simulink model "sst_cllc_dcx"  (R2026b)
settings: Solver=ode23tb  StopTime=param.sim.simlength  FixedStep=tc  MaxStep=param.glb_time.tc
values from neighbouring files (symbols this model uses):
  param = struct()    [init_model.m]
undefined symbols (not defined in the file or in its folder): cllc_dcx_param_example
libraries: fl_lib x144, nesl_utility x71, mos_simple_2th_lib x8, discrete_time_low_pass_filter x2, lithium_ion_battery x1, cllc_dcx x1, single_phase_transformer x1, dab_single_phase_pwm_modulator x1, ee_lib x1
(part 2 of 4)

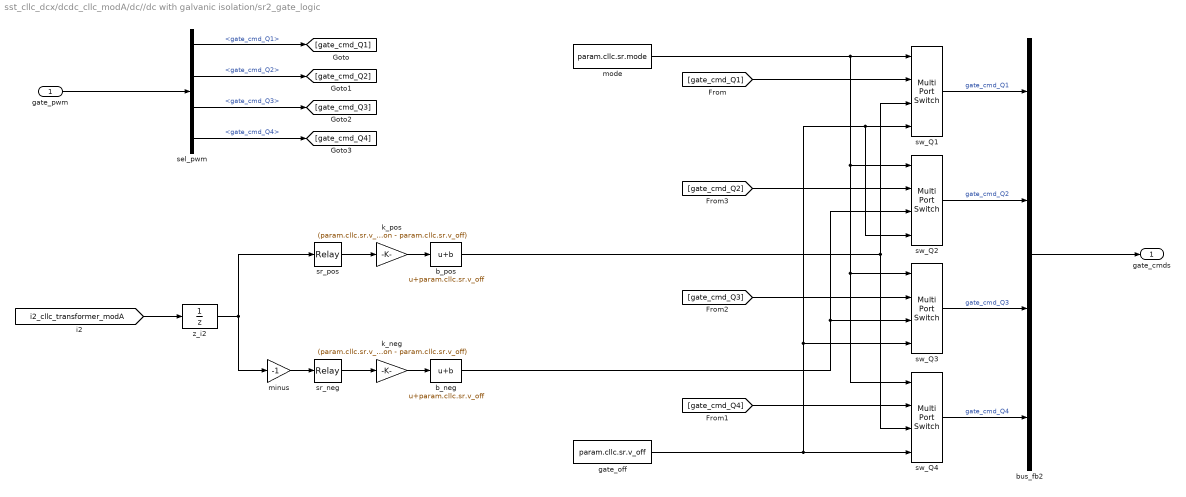
== system sst_cllc_dcx/dcdc_cllc_modA/dc//dc with galvanic isolation/sr2_gate_logic ==
  gate_pwm : Inport
  b_neg : Bias  Bias=param.cllc.sr.v_off  SaturateOnIntegerOverflow=off
  b_pos : Bias  Bias=param.cllc.sr.v_off  SaturateOnIntegerOverflow=off
  bus_fb2 : BusCreator  Inputs=4
  gate_off : Constant  Value=param.cllc.sr.v_off
  k_neg : Gain  Gain=(param.cllc.sr.v_on - param.cllc.sr.v_off)
  k_pos : Gain  Gain=(param.cllc.sr.v_on - param.cllc.sr.v_off)
  minus : Gain  Gain=-1
  mode : Constant  Value=param.cllc.sr.mode
  sel_pwm : BusSelector  OutputSignals=gate_cmd_Q1,gate_cmd_Q2,gate_cmd_Q3,gate_cmd_Q4
  sr_neg : Relay  OnSwitchValue=param.cllc.sr.i_on  OffSwitchValue=param.cllc.sr.i_off
  sr_pos : Relay  OnSwitchValue=param.cllc.sr.i_on  OffSwitchValue=param.cllc.sr.i_off
  sw_Q{1..4} (4 alike) : MultiPortSwitch  DataPortOrder=Zero-based contiguous  zeroidx=on  SaturateOnIntegerOverflow=off  InputSameDT=off
  z_i2 : UnitDelay  SampleTime=param.glb_time.tc
  gate_cmds : Outport
  wires:
  gate_pwm/1 -> sel_pwm/1
  [i2_cllc_transformer_modA] -> z_i2/1
  z_i2/1 -> sr_pos/1, minus/1
  minus/1 -> sr_neg/1
  sr_pos/1 -> k_pos/1
  k_pos/1 -> b_pos/1
  sr_neg/1 -> k_neg/1
  k_neg/1 -> b_neg/1
  mode/1 -> sw_Q1/1, sw_Q2/1, sw_Q3/1, sw_Q4/1
  [gate_cmd_Q1] -> sw_Q1/2
  b_pos/1 -> sw_Q4/3, sw_Q1/3
  gate_off/1 -> sw_Q3/4, sw_Q1/4, sw_Q2/4, sw_Q4/4
  sw_Q1/1 -> bus_fb2/1  "gate_cmd_Q1"
  [gate_cmd_Q2] -> sw_Q2/2
  b_neg/1 -> sw_Q3/3, sw_Q2/3
  sw_Q2/1 -> bus_fb2/2  "gate_cmd_Q2"
  [gate_cmd_Q3] -> sw_Q3/2
  sw_Q3/1 -> bus_fb2/3  "gate_cmd_Q3"
  [gate_cmd_Q4] -> sw_Q4/2
  sw_Q4/1 -> bus_fb2/4  "gate_cmd_Q4"
  bus_fb2/1 -> gate_cmds/1
  sel_pwm/1 -> [gate_cmd_Q1]  "<gate_cmd_Q1>"
  sel_pwm/2 -> [gate_cmd_Q2]  "<gate_cmd_Q2>"
  sel_pwm/3 -> [gate_cmd_Q3]  "<gate_cmd_Q3>"
  sel_pwm/4 -> [gate_cmd_Q4]  "<gate_cmd_Q4>"

== system sst_cllc_dcx/dcdc_cllc_modA/input_current_control/input_current_control ==
  current_input_pu : Inport
  local_time : Inport  Port=2
  Trigger : TriggerPort  VariantControl=(inherit)  PortDimensions=1
  Gain : Gain  Gain=-1
  Gain1 : Gain  Gain=-1
  LLC_current_input_tracking : Scope  NumInputPorts=4
      settings: ActiveDisplayYMinimum=-0.41147300652049457  ActiveDisplayYMaximum=1.0697728708256782  DataLoggingVariableName=ScopeData12
  Quantizer : Quantizer  QuantizationInterval=param.meas.adc12_quantization
  Step : Step  InitialValue=1  FinalValue=-1
  To Workspace1 : ToWorkspace  VariableName=cllc_input_current_ref_sim  SampleTime=-1
      settings: MaxDataPoints=param.glb_time.Ns_cllc
  To Workspace14 : ToWorkspace  VariableName=time_ts_sim  SampleTime=-1
      settings: MaxDataPoints=param.glb_time.Ns_cllc
  To Workspace2 : ToWorkspace  VariableName=cllc_input_current_sim  SampleTime=-1
      settings: MaxDataPoints=param.glb_time.Ns_cllc
  To Workspace3 : ToWorkspace  VariableName=cllc_current_ctrl_output_sim  SampleTime=-1
      settings: MaxDataPoints=param.glb_time.Ns_cllc
  Unit Delay2 : UnitDelay  SampleTime=-1
  Zero-Order Hold1 : ZeroOrderHold  SampleTime=-1
  Zero-Order Hold2 : ZeroOrderHold  SampleTime=-1
  current_control : Subsystem
  discrete-time-low-pass-filter : discrete_time_low_pass_filter/discrete-time-low-pass-filter  tau=0.025  ts=param.glb_time.ts_cllc
  discrete-time-low-pass-filter1 : discrete_time_low_pass_filter/discrete-time-low-pass-filter  tau=0.025  ts=param.glb_time.ts_cllc
  ictrl_out : Outport
  wires:
  Unit Delay2/1 -> To Workspace3/1, LLC_current_input_tracking/3, ictrl_out/1  "current_ctrl_output"
  current_control/1(ctrli_out) -> Gain/1
  Quantizer/1 -> Zero-Order Hold2/1
  current_input_pu/1 -> Quantizer/1
  Zero-Order Hold2/1 -> LLC_current_input_tracking/2, To Workspace2/1, current_control/2(iout), LLC_current_input_tracking/4  "i_dc_input"
  Gain/1 -> Unit Delay2/1
  local_time/1 -> Zero-Order Hold1/1
  Zero-Order Hold1/1 -> To Workspace14/1
  Step/1 -> Gain1/1
  discrete-time-low-pass-filter/1 -> LLC_current_input_tracking/1, To Workspace1/1, current_control/1(iout_ref)  "current_input_ref"
  Gain1/1 -> discrete-time-low-pass-filter/1

== system sst_cllc_dcx/dcdc_cllc_modA/input_current_control/modulator ==
  phase_displacement : Inport
  Constant1 : Constant  Value=0.5
  Constant2 : Constant  Value=0.5
  Constant3 : Constant  Value=0.02
  dab_single_phase_pwm_modulator : dab_single_phase_pwm_modulator/dab_single_phase_pwm_modulator  fPWM_DAB=param.glb_time.fPWM_CLLC  m_up=1  m_low=0  dead_time_DAB=param.glb_time.dead_time_CLLC  pos_cmd_gate=18  neg_cmd_gate=-3  polarity=-1  tc=param.glb_time.tc  max_phase_displacement=pi/2  trgo_double_update=param.glb_time.TRGO_CLLC_double_update
  gate_cmds : Outport
  tag scope: TRGO=global
  wires:
  dab_single_phase_pwm_modulator/2 -> gate_cmds/1
  Constant2/1 -> dab_single_phase_pwm_modulator/3
  dab_single_phase_pwm_modulator/1 -> [TRGO]
  Constant1/1 -> dab_single_phase_pwm_modulator/2
  [time_cllc_module_1] -> dab_single_phase_pwm_modulator/1
  Constant3/1 -> dab_single_phase_pwm_modulator/4

== system sst_cllc_dcx/dcdc_cllc_modA/input_current_control/normalization ==
  in : Inport
  1/Ti3 : Gain  Gain=1/param.cllc.hw.Idc_FS  OutDataTypeStr=double  SaturateOnIntegerOverflow=on  ParamDataTypeStr=Inherit: Same as input
  out_pu : Outport
  wires:
  in/1 -> 1/Ti3/1
  1/Ti3/1 -> out_pu/1

== system sst_cllc_dcx/dcdc_cllc_modA/dc//dc with galvanic isolation/full-bridge 1/full-full_bridge_ssc_mosfet_based ==
  gate_commands : Inport
  data_measure : Subsystem
  full_bridge_ssc_mosfet_based : Subsystem  mask{mass_heatsink_m=param.thermal.heatsink.no_weight, specific_heat_m=param.thermal.heatsink.cp, rth_mosfet_HA_m=param.thermal.heatsink.Rth_mosfet_HA, rth_mosfet_JH_m=param.cllc.mosfet.Rth_mosfet_JH, Rds_on_m=param.cllc.mosfet.Rds_on, Vth_m=param.cllc.mosfet.Vth, Eon_m=param.cllc.mosfet.Eon, Eoff_m=param.cllc.mosfet.Eoff, Voff_sw_loss_m=param.cllc.mosfet.Voff_sw_losses, Ion_sw_loss_m=param.cllc.mosfet.Ion_sw_losses, Vdon_diode_m=param.cllc.mosfet.Vdon_diode, Rdon_diode_m=param.cllc.mosfet.Rds_on, JunctionTermalMass_m=param.cllc.mosfet.JunctionTermalMass, Tambient_m=param.thermal.Tambient, DThs_init_m=param.thermal.DThs_init, Csnubber_m=param.cllc.mosfet.Csnubber_zvs, Rsnubber_m=param.cllc.mosfet.Rsnubber_zvs}
      mask prompts: mass_heatsink_m "Mass Heatsink (kg)"; specific_heat_m "Specific Heat (J/K/kg)"; rth_mosfet_HA_m "Thermal Resistance HA (K/W)"; rth_mosfet_JH_m "Thermal Resistance JH (K/W)"; Rds_on_m "Rds_on (Ohm)"; Vth_m "Vth (V)"; Eon_m "Eon (J)"; Eoff_m "Eoff (J)"; Voff_sw_loss_m "Voff_sw_loss (V)"; Ion_sw_loss_m "Ion_sw_loss (A)"; Vdon_diode_m "Vdon_diode (V)"; Rdon_diode_m "Rdon_diode (Ohm)"; JunctionTermalMass_m "JunctionTermalMass (J/K)"; Tambient_m "Tambient (degC)"; DThs_init_m "DThs_init (degC)"; Csnubber_m "Csnubber (F)"; Rsnubber_m "Rsnubber (Ohm)"
  udc(+) : PMIOPort  Side=Left
  udc(-) : PMIOPort  Port=2  Side=Left
  uac(+) : PMIOPort  Port=3  Side=Right
  uac(-) : PMIOPort  Port=4  Side=Right
  wires:
  full_bridge_ssc_mosfet_based/1(m) -> data_measure/1(m)
  gate_commands/1 -> full_bridge_ssc_mosfet_based/1(gate_commands)
  connections:
  full_bridge_ssc_mosfet_based/LConn2 -- udc(-)/RConn1
  full_bridge_ssc_mosfet_based/LConn1 -- udc(+)/RConn1
  full_bridge_ssc_mosfet_based/RConn2 -- uac(-)/RConn1
  full_bridge_ssc_mosfet_based/RConn1 -- uac(+)/RConn1

== system sst_cllc_dcx/dcdc_cllc_modA/dc//dc with galvanic isolation/full-bridge 2/full_bridge_ssc_mosfet_based ==
  gate_commands : Inport
  data_measure : Subsystem
  full_bridge_ssc_mosfet_based : Subsystem  mask{mass_heatsink_m=param.thermal.heatsink.no_weight, specific_heat_m=param.thermal.heatsink.cp, rth_mosfet_HA_m=param.thermal.heatsink.Rth_mosfet_HA, rth_mosfet_JH_m=param.cllc.mosfet_sr.Rth_mosfet_JH, Rds_on_m=param.cllc.mosfet_sr.Rds_on, Vth_m=param.cllc.mosfet_sr.Vth, Eon_m=param.cllc.mosfet_sr.Eon, Eoff_m=param.cllc.mosfet_sr.Eoff, Voff_sw_loss_m=param.cllc.mosfet_sr.Voff_sw_losses, Ion_sw_loss_m=param.cllc.mosfet_sr.Ion_sw_losses, Vdon_diode_m=param.cllc.mosfet_sr.Vdon_diode, Rdon_diode_m=param.cllc.mosfet_sr.Rds_on, JunctionTermalMass_m=param.cllc.mosfet_sr.JunctionTermalMass, Tambient_m=param.thermal.Tambient, DThs_init_m=param.thermal.DThs_init, Csnubber_m=param.cllc.mosfet_sr.Csnubber_zvs, Rsnubber_m=param.cllc.mosfet_sr.Rsnubber_zvs}
      mask prompts: mass_heatsink_m "Mass Heatsink (kg)"; specific_heat_m "Specific Heat (J/K/kg)"; rth_mosfet_HA_m "Thermal Resistance HA (K/W)"; rth_mosfet_JH_m "Thermal Resistance JH (K/W)"; Rds_on_m "Rds_on (Ohm)"; Vth_m "Vth (V)"; Eon_m "Eon (J)"; Eoff_m "Eoff (J)"; Voff_sw_loss_m "Voff_sw_loss (V)"; Ion_sw_loss_m "Ion_sw_loss (A)"; Vdon_diode_m "Vdon_diode (V)"; Rdon_diode_m "Rdon_diode (Ohm)"; JunctionTermalMass_m "JunctionTermalMass (J/K)"; Tambient_m "Tambient (degC)"; DThs_init_m "DThs_init (degC)"; Csnubber_m "Csnubber (F)"; Rsnubber_m "Rsnubber (Ohm)"
  udc(+) : PMIOPort  Side=Left
  udc(-) : PMIOPort  Port=2  Side=Left
  uac(+) : PMIOPort  Port=3  Side=Right
  uac(-) : PMIOPort  Port=4  Side=Right
  wires:
  full_bridge_ssc_mosfet_based/1(m) -> data_measure/1(m)
  gate_commands/1 -> full_bridge_ssc_mosfet_based/1(gate_commands)
  connections:
  full_bridge_ssc_mosfet_based/LConn2 -- udc(-)/RConn1
  full_bridge_ssc_mosfet_based/LConn1 -- udc(+)/RConn1
  full_bridge_ssc_mosfet_based/RConn2 -- uac(-)/RConn1
  full_bridge_ssc_mosfet_based/RConn1 -- uac(+)/RConn1

== system sst_cllc_dcx/dcdc_cllc_modA/input_current_control/input_current_control/current_control ==
  iout_ref : Inport
  iout : Inport  Port=2
  Sum2 : Sum  Inputs=+-  OutDataTypeStr=double  AccumDataTypeStr=double  SaturateOnIntegerOverflow=on
  iout_ctrl : Subsystem
  ctrli_out : Outport
  wires:
  iout_ctrl/1(phase_shift) -> ctrli_out/1
  iout/1 -> Sum2/2
  iout_ref/1 -> Sum2/1
  Sum2/1 -> iout_ctrl/1(i_tilde)

== system sst_cllc_dcx/dcdc_cllc_modA/dc//dc with galvanic isolation/full-bridge 1/full-full_bridge_ssc_mosfet_based/data_measure ==
  m : Inport
  Bus Selector : BusSelector  OutputSignals=mosfet_ploss_Q1,mosfet_voltage_Q1,mosfet_current_Q1,mosfet_JH_temp_Q1,mosfet_HA_temp_Q1
  Bus Selector1 : BusSelector  OutputSignals=mosfet_ploss_Q2,mosfet_voltage_Q2,mosfet_current_Q2,mosfet_JH_temp_Q2,mosfet_HA_temp_Q2
  tag scope: inverter_1_cllc_mosfet_zvs_modA=global, mosfet_zvs_HA_temp_cllc_Q1=global, mosfet_zvs_HA_temp_cllc_Q2=global, mosfet_zvs_JH_temp_cllc_Q1=global, mosfet_zvs_JH_temp_cllc_Q2=global, mosfet_zvs_ids_cllc_Q1=global, mosfet_zvs_ids_cllc_Q2=global, mosfet_zvs_plosses_cllc_Q1=global, mosfet_zvs_plosses_cllc_Q2=global, mosfet_zvs_uds_cllc_Q1=global, mosfet_zvs_uds_cllc_Q2=global
  wires:
  Bus Selector/1 -> [mosfet_zvs_plosses_cllc_Q1]  "<mosfet_ploss_Q1>"
  Bus Selector1/3 -> [mosfet_zvs_ids_cllc_Q2]  "<mosfet_current_Q2>"
  Bus Selector1/2 -> [mosfet_zvs_uds_cllc_Q2]  "<mosfet_voltage_Q2>"
  Bus Selector1/5 -> [mosfet_zvs_HA_temp_cllc_Q2]  "<mosfet_HA_temp_Q2>"
  Bus Selector/4 -> [mosfet_zvs_JH_temp_cllc_Q1]  "<mosfet_JH_temp_Q1>"
  Bus Selector/5 -> [mosfet_zvs_HA_temp_cllc_Q1]  "<mosfet_HA_temp_Q1>"
  Bus Selector1/4 -> [mosfet_zvs_JH_temp_cllc_Q2]  "<mosfet_JH_temp_Q2>"
  Bus Selector/3 -> [mosfet_zvs_ids_cllc_Q1]  "<mosfet_current_Q1>"
  Bus Selector/2 -> [mosfet_zvs_uds_cllc_Q1]  "<mosfet_voltage_Q1>"
  Bus Selector1/1 -> [mosfet_zvs_plosses_cllc_Q2]  "<mosfet_ploss_Q2>"
  m/1 -> Bus Selector/1, Bus Selector1/1, [inverter_1_cllc_mosfet_zvs_modA]

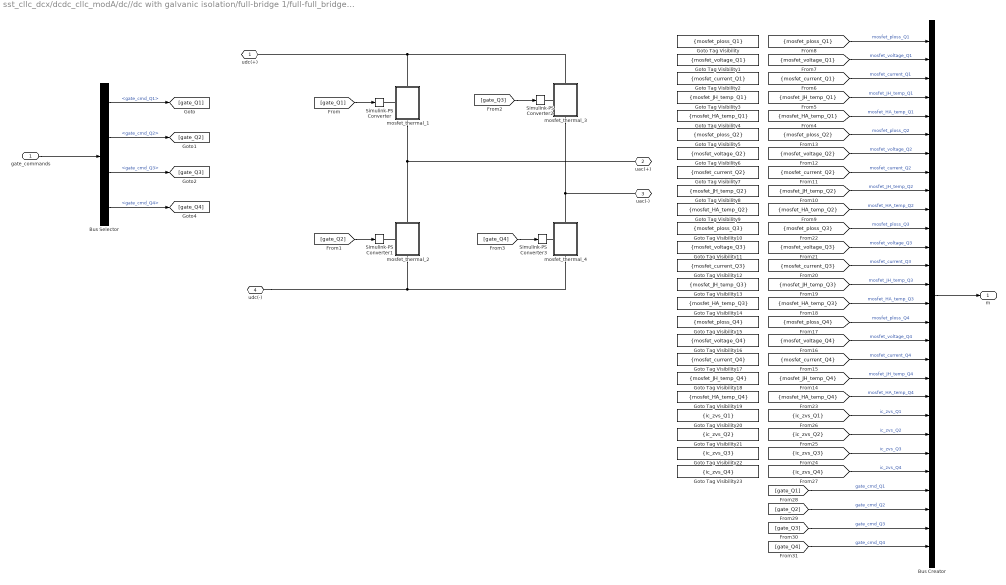
== system sst_cllc_dcx/dcdc_cllc_modA/dc//dc with galvanic isolation/full-bridge 1/full-full_bridge_ssc_mosfet_based/full_bridge_ssc_mosfet_based ==
  gate_commands : Inport
  Bus Creator : BusCreator  Inputs=28
  Bus Selector : BusSelector  OutputSignals=gate_cmd_Q1,gate_cmd_Q2,gate_cmd_Q3,gate_cmd_Q4
  Goto Tag Visibility : GotoTagVisibility  GotoTag=mosfet_ploss_Q1
  Goto Tag Visibility1 : GotoTagVisibility  GotoTag=mosfet_voltage_Q1
  Goto Tag Visibility10 : GotoTagVisibility  GotoTag=mosfet_ploss_Q3
  Goto Tag Visibility11 : GotoTagVisibility  GotoTag=mosfet_voltage_Q3
  Goto Tag Visibility12 : GotoTagVisibility  GotoTag=mosfet_current_Q3
  Goto Tag Visibility13 : GotoTagVisibility  GotoTag=mosfet_JH_temp_Q3
  Goto Tag Visibility14 : GotoTagVisibility  GotoTag=mosfet_HA_temp_Q3
  Goto Tag Visibility15 : GotoTagVisibility  GotoTag=mosfet_ploss_Q4
  Goto Tag Visibility16 : GotoTagVisibility  GotoTag=mosfet_voltage_Q4
  Goto Tag Visibility17 : GotoTagVisibility  GotoTag=mosfet_current_Q4
  Goto Tag Visibility18 : GotoTagVisibility  GotoTag=mosfet_JH_temp_Q4
  Goto Tag Visibility19 : GotoTagVisibility  GotoTag=mosfet_HA_temp_Q4
  Goto Tag Visibility2 : GotoTagVisibility  GotoTag=mosfet_current_Q1
  Goto Tag Visibility20 : GotoTagVisibility  GotoTag=ic_zvs_Q1
  Goto Tag Visibility21 : GotoTagVisibility  GotoTag=ic_zvs_Q2
  Goto Tag Visibility22 : GotoTagVisibility  GotoTag=ic_zvs_Q3
  Goto Tag Visibility23 : GotoTagVisibility  GotoTag=ic_zvs_Q4
  Goto Tag Visibility3 : GotoTagVisibility  GotoTag=mosfet_JH_temp_Q1
  Goto Tag Visibility4 : GotoTagVisibility  GotoTag=mosfet_HA_temp_Q1
  Goto Tag Visibility5 : GotoTagVisibility  GotoTag=mosfet_ploss_Q2
  Goto Tag Visibility6 : GotoTagVisibility  GotoTag=mosfet_voltage_Q2
  Goto Tag Visibility7 : GotoTagVisibility  GotoTag=mosfet_current_Q2
  Goto Tag Visibility8 : GotoTagVisibility  GotoTag=mosfet_JH_temp_Q2
  Goto Tag Visibility9 : GotoTagVisibility  GotoTag=mosfet_HA_temp_Q2
  Simulink-PS Converter{,1..3} (4 alike) : nesl_utility/Simulink-PS Converter  PhysicalDomain=network_engine_domain  SubClassName=ps_input  LeftPortType=input  RightPortType=output  PseudoPeriodic=off  Frequencies=[]  NoiseDistribution=none  NoiseParameters=[]  Unit=V  AffineConversion=off  FilteringAndDerivatives=provide  SimscapeFilterOrder=1  InputFilterTimeConstant=0.001  UdotUserProvided=0
  mosfet_thermal_1 : Subsystem
      settings: PortSchema="{\"entries\":[{\"content\":{\"sides\":[{\"content\":{\"connectorIds\":[\"LConn1\"]},\"type\":\"ConnectorPlacement.EquallySpacedRectSide\",\"uuid\":\"9277da8d-d460-43e6-8478-dd662f15d226\"},{\"content\":{\"connectorIds\":[],\"side\":\"RIGHT\"},\"type\":\"ConnectorPlacement.EquallySpacedRectSide\",\"uuid\":\"a7ece396-f1d9-4f4f-a05b-db1fc65d6e1d\"},{\"content\":{\"connectorIds\":[\"LConn2\"],\"side\":\"TOP\"},\"type\":\"ConnectorPlacement.EquallySpacedRectSide\",\"uuid\":\"fdd70777-e9cf-4317-afb6-cae87f75d5b0\"},{\"content\":{\"connectorIds\":[\"RConn1\"],\"side\":\"BOTTOM\"},\"type\":\"ConnectorPlacement.EquallySpacedRectSide\",\"uuid\":\"2353ed68-b1a1-4775-9ca9-31e268d5443b\"}]},\"type\":\"ConnectorPlacement.EquallySpacedConnector\",\"uuid\":\"d5479f4c-4e65-4791-adcb-73df11f88590\"}],\"packageUris\":[\"http://schema.mathworks.com/mf0/Connector/R2020b\"],\"version\":\"1.0\"}"
  mosfet_thermal_2 : Subsystem
      settings: PortSchema="{\"entries\":[{\"content\":{\"sides\":[{\"content\":{\"connectorIds\":[\"LConn1\"]},\"type\":\"ConnectorPlacement.EquallySpacedRectSide\",\"uuid\":\"9277da8d-d460-43e6-8478-dd662f15d226\"},{\"content\":{\"connectorIds\":[],\"side\":\"RIGHT\"},\"type\":\"ConnectorPlacement.EquallySpacedRectSide\",\"uuid\":\"a7ece396-f1d9-4f4f-a05b-db1fc65d6e1d\"},{\"content\":{\"connectorIds\":[\"LConn2\"],\"side\":\"TOP\"},\"type\":\"ConnectorPlacement.EquallySpacedRectSide\",\"uuid\":\"fdd70777-e9cf-4317-afb6-cae87f75d5b0\"},{\"content\":{\"connectorIds\":[\"RConn1\"],\"side\":\"BOTTOM\"},\"type\":\"ConnectorPlacement.EquallySpacedRectSide\",\"uuid\":\"2353ed68-b1a1-4775-9ca9-31e268d5443b\"}]},\"type\":\"ConnectorPlacement.EquallySpacedConnector\",\"uuid\":\"d5479f4c-4e65-4791-adcb-73df11f88590\"}],\"packageUris\":[\"http://schema.mathworks.com/mf0/Connector/R2020b\"],\"version\":\"1.0\"}"
  mosfet_thermal_3 : Subsystem
      settings: PortSchema="{\"entries\":[{\"content\":{\"sides\":[{\"content\":{\"connectorIds\":[\"LConn1\"]},\"type\":\"ConnectorPlacement.EquallySpacedRectSide\",\"uuid\":\"9277da8d-d460-43e6-8478-dd662f15d226\"},{\"content\":{\"connectorIds\":[],\"side\":\"RIGHT\"},\"type\":\"ConnectorPlacement.EquallySpacedRectSide\",\"uuid\":\"a7ece396-f1d9-4f4f-a05b-db1fc65d6e1d\"},{\"content\":{\"connectorIds\":[\"LConn2\"],\"side\":\"TOP\"},\"type\":\"ConnectorPlacement.EquallySpacedRectSide\",\"uuid\":\"fdd70777-e9cf-4317-afb6-cae87f75d5b0\"},{\"content\":{\"connectorIds\":[\"RConn1\"],\"side\":\"BOTTOM\"},\"type\":\"ConnectorPlacement.EquallySpacedRectSide\",\"uuid\":\"2353ed68-b1a1-4775-9ca9-31e268d5443b\"}]},\"type\":\"ConnectorPlacement.EquallySpacedConnector\",\"uuid\":\"d5479f4c-4e65-4791-adcb-73df11f88590\"}],\"packageUris\":[\"http://schema.mathworks.com/mf0/Connector/R2020b\"],\"version\":\"1.0\"}"
  mosfet_thermal_4 : Subsystem
      settings: PortSchema="{\"entries\":[{\"content\":{\"sides\":[{\"content\":{\"connectorIds\":[\"LConn1\"]},\"type\":\"ConnectorPlacement.EquallySpacedRectSide\",\"uuid\":\"9277da8d-d460-43e6-8478-dd662f15d226\"},{\"content\":{\"connectorIds\":[],\"side\":\"RIGHT\"},\"type\":\"ConnectorPlacement.EquallySpacedRectSide\",\"uuid\":\"a7ece396-f1d9-4f4f-a05b-db1fc65d6e1d\"},{\"content\":{\"connectorIds\":[\"LConn2\"],\"side\":\"TOP\"},\"type\":\"ConnectorPlacement.EquallySpacedRectSide\",\"uuid\":\"fdd70777-e9cf-4317-afb6-cae87f75d5b0\"},{\"content\":{\"connectorIds\":[\"RConn1\"],\"side\":\"BOTTOM\"},\"type\":\"ConnectorPlacement.EquallySpacedRectSide\",\"uuid\":\"2353ed68-b1a1-4775-9ca9-31e268d5443b\"}]},\"type\":\"ConnectorPlacement.EquallySpacedConnector\",\"uuid\":\"d5479f4c-4e65-4791-adcb-73df11f88590\"}],\"packageUris\":[\"http://schema.mathworks.com/mf0/Connector/R2020b\"],\"version\":\"1.0\"}"
  udc(+) : PMIOPort  Side=Left
  uac(+) : PMIOPort  Port=2  Side=Right
  uac(-) : PMIOPort  Port=3  Side=Right
  udc(-) : PMIOPort  Port=4  Side=Left
  m : Outport
  wires:
  [gate_Q4] -> Bus Creator/28  "gate_cmd_Q4"
  [gate_Q3] -> Bus Creator/27  "gate_cmd_Q3"
  [gate_Q2] -> Bus Creator/26  "gate_cmd_Q2"
  [gate_Q1] -> Bus Creator/25  "gate_cmd_Q1"
  [ic_zvs_Q4] -> Bus Creator/24  "ic_zvs_Q4"
  [ic_zvs_Q3] -> Bus Creator/23  "ic_zvs_Q3"
  [ic_zvs_Q2] -> Bus Creator/22  "ic_zvs_Q2"
  [ic_zvs_Q1] -> Bus Creator/21  "ic_zvs_Q1"
  Bus Creator/1 -> m/1
  [mosfet_HA_temp_Q4] -> Bus Creator/20  "mosfet_HA_temp_Q4"
  [mosfet_JH_temp_Q4] -> Bus Creator/19  "mosfet_JH_temp_Q4"
  [mosfet_current_Q4] -> Bus Creator/18  "mosfet_current_Q4"
  [mosfet_voltage_Q4] -> Bus Creator/17  "mosfet_voltage_Q4"
  [mosfet_ploss_Q4] -> Bus Creator/16  "mosfet_ploss_Q4"
  [mosfet_HA_temp_Q3] -> Bus Creator/15  "mosfet_HA_temp_Q3"
  [mosfet_JH_temp_Q3] -> Bus Creator/14  "mosfet_JH_temp_Q3"
  [mosfet_current_Q3] -> Bus Creator/13  "mosfet_current_Q3"
  [mosfet_voltage_Q3] -> Bus Creator/12  "mosfet_voltage_Q3"
  [mosfet_ploss_Q3] -> Bus Creator/11  "mosfet_ploss_Q3"
  [mosfet_HA_temp_Q2] -> Bus Creator/10  "mosfet_HA_temp_Q2"
  [mosfet_JH_temp_Q2] -> Bus Creator/9  "mosfet_JH_temp_Q2"
  [mosfet_current_Q2] -> Bus Creator/8  "mosfet_current_Q2"
  [mosfet_voltage_Q2] -> Bus Creator/7  "mosfet_voltage_Q2"
  [mosfet_ploss_Q2] -> Bus Creator/6  "mosfet_ploss_Q2"
  [mosfet_HA_temp_Q1] -> Bus Creator/5  "mosfet_HA_temp_Q1"
  [mosfet_JH_temp_Q1] -> Bus Creator/4  "mosfet_JH_temp_Q1"
  [mosfet_current_Q1] -> Bus Creator/3  "mosfet_current_Q1"
  [mosfet_voltage_Q1] -> Bus Creator/2  "mosfet_voltage_Q1"
  [mosfet_ploss_Q1] -> Bus Creator/1  "mosfet_ploss_Q1"
  [gate_Q3] -> Simulink-PS Converter2/1
  Bus Selector/2 -> [gate_Q2]  "<gate_cmd_Q2>"
  Bus Selector/1 -> [gate_Q1]  "<gate_cmd_Q1>"
  Bus Selector/3 -> [gate_Q3]  "<gate_cmd_Q3>"
  [gate_Q4] -> Simulink-PS Converter3/1
  [gate_Q2] -> Simulink-PS Converter1/1
  [gate_Q1] -> Simulink-PS Converter/1
  Bus Selector/4 -> [gate_Q4]  "<gate_cmd_Q4>"
  gate_commands/1 -> Bus Selector/1
  connections:
  mosfet_thermal_1/LConn1 -- Simulink-PS Converter/RConn1
  mosfet_thermal_3/LConn2 -- udc(+)/RConn1 -- mosfet_thermal_1/LConn2
  mosfet_thermal_4/RConn1 -- udc(-)/RConn1 -- mosfet_thermal_2/RConn1
  mosfet_thermal_2/LConn2 -- mosfet_thermal_1/RConn1 -- uac(+)/RConn1
  mosfet_thermal_3/LConn1 -- Simulink-PS Converter2/RConn1
  mosfet_thermal_4/LConn2 -- uac(-)/RConn1 -- mosfet_thermal_3/RConn1
  mosfet_thermal_2/LConn1 -- Simulink-PS Converter1/RConn1
  mosfet_thermal_4/LConn1 -- Simulink-PS Converter3/RConn1

== system sst_cllc_dcx/dcdc_cllc_modA/dc//dc with galvanic isolation/full-bridge 2/full_bridge_ssc_mosfet_based/data_measure ==
  m : Inport
  Bus Selector : BusSelector  OutputSignals=mosfet_ploss_Q1,mosfet_voltage_Q1,mosfet_current_Q1,mosfet_JH_temp_Q1,mosfet_HA_temp_Q1
  Bus Selector1 : BusSelector  OutputSignals=mosfet_ploss_Q2,mosfet_voltage_Q2,mosfet_current_Q2,mosfet_JH_temp_Q2,mosfet_HA_temp_Q2
  tag scope: inverter_2_cllc_mosfet_zvs_modA=global, mosfet_zvs_HA_temp_cllc_Q5=global, mosfet_zvs_HA_temp_cllc_Q6=global, mosfet_zvs_JH_temp_cllc_Q5=global, mosfet_zvs_JH_temp_cllc_Q6=global, mosfet_zvs_ids_cllc_Q5=global, mosfet_zvs_ids_cllc_Q6=global, mosfet_zvs_plosses_cllc_Q5=global, mosfet_zvs_plosses_cllc_Q6=global, mosfet_zvs_uds_cllc_Q5=global, mosfet_zvs_uds_cllc_Q6=global
  wires:
  Bus Selector/1 -> [mosfet_zvs_plosses_cllc_Q5]  "<mosfet_ploss_Q1>"
  Bus Selector1/3 -> [mosfet_zvs_ids_cllc_Q6]  "<mosfet_current_Q2>"
  Bus Selector1/2 -> [mosfet_zvs_uds_cllc_Q6]  "<mosfet_voltage_Q2>"
  Bus Selector1/5 -> [mosfet_zvs_HA_temp_cllc_Q6]  "<mosfet_HA_temp_Q2>"
  Bus Selector/4 -> [mosfet_zvs_JH_temp_cllc_Q5]  "<mosfet_JH_temp_Q1>"
  Bus Selector/5 -> [mosfet_zvs_HA_temp_cllc_Q5]  "<mosfet_HA_temp_Q1>"
  Bus Selector1/4 -> [mosfet_zvs_JH_temp_cllc_Q6]  "<mosfet_JH_temp_Q2>"
  Bus Selector/3 -> [mosfet_zvs_ids_cllc_Q5]  "<mosfet_current_Q1>"
  Bus Selector/2 -> [mosfet_zvs_uds_cllc_Q5]  "<mosfet_voltage_Q1>"
  Bus Selector1/1 -> [mosfet_zvs_plosses_cllc_Q6]  "<mosfet_ploss_Q2>"
  m/1 -> Bus Selector/1, Bus Selector1/1, [inverter_2_cllc_mosfet_zvs_modA]

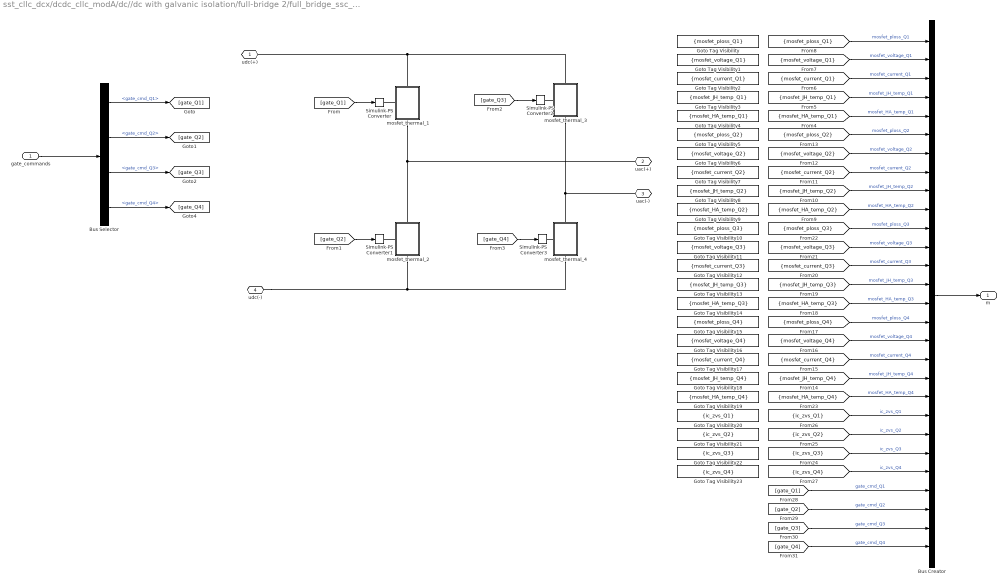
== system sst_cllc_dcx/dcdc_cllc_modA/dc//dc with galvanic isolation/full-bridge 2/full_bridge_ssc_mosfet_based/full_bridge_ssc_mosfet_based ==
  gate_commands : Inport
  Bus Creator : BusCreator  Inputs=28
  Bus Selector : BusSelector  OutputSignals=gate_cmd_Q1,gate_cmd_Q2,gate_cmd_Q3,gate_cmd_Q4
  Goto Tag Visibility : GotoTagVisibility  GotoTag=mosfet_ploss_Q1
  Goto Tag Visibility1 : GotoTagVisibility  GotoTag=mosfet_voltage_Q1
  Goto Tag Visibility10 : GotoTagVisibility  GotoTag=mosfet_ploss_Q3
  Goto Tag Visibility11 : GotoTagVisibility  GotoTag=mosfet_voltage_Q3
  Goto Tag Visibility12 : GotoTagVisibility  GotoTag=mosfet_current_Q3
  Goto Tag Visibility13 : GotoTagVisibility  GotoTag=mosfet_JH_temp_Q3
  Goto Tag Visibility14 : GotoTagVisibility  GotoTag=mosfet_HA_temp_Q3
  Goto Tag Visibility15 : GotoTagVisibility  GotoTag=mosfet_ploss_Q4
  Goto Tag Visibility16 : GotoTagVisibility  GotoTag=mosfet_voltage_Q4
  Goto Tag Visibility17 : GotoTagVisibility  GotoTag=mosfet_current_Q4
  Goto Tag Visibility18 : GotoTagVisibility  GotoTag=mosfet_JH_temp_Q4
  Goto Tag Visibility19 : GotoTagVisibility  GotoTag=mosfet_HA_temp_Q4
  Goto Tag Visibility2 : GotoTagVisibility  GotoTag=mosfet_current_Q1
  Goto Tag Visibility20 : GotoTagVisibility  GotoTag=ic_zvs_Q1
  Goto Tag Visibility21 : GotoTagVisibility  GotoTag=ic_zvs_Q2
  Goto Tag Visibility22 : GotoTagVisibility  GotoTag=ic_zvs_Q3
  Goto Tag Visibility23 : GotoTagVisibility  GotoTag=ic_zvs_Q4
  Goto Tag Visibility3 : GotoTagVisibility  GotoTag=mosfet_JH_temp_Q1
  Goto Tag Visibility4 : GotoTagVisibility  GotoTag=mosfet_HA_temp_Q1
  Goto Tag Visibility5 : GotoTagVisibility  GotoTag=mosfet_ploss_Q2
  Goto Tag Visibility6 : GotoTagVisibility  GotoTag=mosfet_voltage_Q2
  Goto Tag Visibility7 : GotoTagVisibility  GotoTag=mosfet_current_Q2
  Goto Tag Visibility8 : GotoTagVisibility  GotoTag=mosfet_JH_temp_Q2
  Goto Tag Visibility9 : GotoTagVisibility  GotoTag=mosfet_HA_temp_Q2
  Simulink-PS Converter{,1..3} (4 alike) : nesl_utility/Simulink-PS Converter  PhysicalDomain=network_engine_domain  SubClassName=ps_input  LeftPortType=input  RightPortType=output  PseudoPeriodic=off  Frequencies=[]  NoiseDistribution=none  NoiseParameters=[]  Unit=V  AffineConversion=off  FilteringAndDerivatives=provide  SimscapeFilterOrder=1  InputFilterTimeConstant=0.001  UdotUserProvided=0
  mosfet_thermal_1 : Subsystem
      settings: PortSchema="{\"entries\":[{\"content\":{\"sides\":[{\"content\":{\"connectorIds\":[\"LConn1\"]},\"type\":\"ConnectorPlacement.EquallySpacedRectSide\",\"uuid\":\"9277da8d-d460-43e6-8478-dd662f15d226\"},{\"content\":{\"connectorIds\":[],\"side\":\"RIGHT\"},\"type\":\"ConnectorPlacement.EquallySpacedRectSide\",\"uuid\":\"a7ece396-f1d9-4f4f-a05b-db1fc65d6e1d\"},{\"content\":{\"connectorIds\":[\"LConn2\"],\"side\":\"TOP\"},\"type\":\"ConnectorPlacement.EquallySpacedRectSide\",\"uuid\":\"fdd70777-e9cf-4317-afb6-cae87f75d5b0\"},{\"content\":{\"connectorIds\":[\"RConn1\"],\"side\":\"BOTTOM\"},\"type\":\"ConnectorPlacement.EquallySpacedRectSide\",\"uuid\":\"2353ed68-b1a1-4775-9ca9-31e268d5443b\"}]},\"type\":\"ConnectorPlacement.EquallySpacedConnector\",\"uuid\":\"d5479f4c-4e65-4791-adcb-73df11f88590\"}],\"packageUris\":[\"http://schema.mathworks.com/mf0/Connector/R2020b\"],\"version\":\"1.0\"}"
  mosfet_thermal_2 : Subsystem
      settings: PortSchema="{\"entries\":[{\"content\":{\"sides\":[{\"content\":{\"connectorIds\":[\"LConn1\"]},\"type\":\"ConnectorPlacement.EquallySpacedRectSide\",\"uuid\":\"9277da8d-d460-43e6-8478-dd662f15d226\"},{\"content\":{\"connectorIds\":[],\"side\":\"RIGHT\"},\"type\":\"ConnectorPlacement.EquallySpacedRectSide\",\"uuid\":\"a7ece396-f1d9-4f4f-a05b-db1fc65d6e1d\"},{\"content\":{\"connectorIds\":[\"LConn2\"],\"side\":\"TOP\"},\"type\":\"ConnectorPlacement.EquallySpacedRectSide\",\"uuid\":\"fdd70777-e9cf-4317-afb6-cae87f75d5b0\"},{\"content\":{\"connectorIds\":[\"RConn1\"],\"side\":\"BOTTOM\"},\"type\":\"ConnectorPlacement.EquallySpacedRectSide\",\"uuid\":\"2353ed68-b1a1-4775-9ca9-31e268d5443b\"}]},\"type\":\"ConnectorPlacement.EquallySpacedConnector\",\"uuid\":\"d5479f4c-4e65-4791-adcb-73df11f88590\"}],\"packageUris\":[\"http://schema.mathworks.com/mf0/Connector/R2020b\"],\"version\":\"1.0\"}"
  mosfet_thermal_3 : Subsystem
      settings: PortSchema="{\"entries\":[{\"content\":{\"sides\":[{\"content\":{\"connectorIds\":[\"LConn1\"]},\"type\":\"ConnectorPlacement.EquallySpacedRectSide\",\"uuid\":\"9277da8d-d460-43e6-8478-dd662f15d226\"},{\"content\":{\"connectorIds\":[],\"side\":\"RIGHT\"},\"type\":\"ConnectorPlacement.EquallySpacedRectSide\",\"uuid\":\"a7ece396-f1d9-4f4f-a05b-db1fc65d6e1d\"},{\"content\":{\"connectorIds\":[\"LConn2\"],\"side\":\"TOP\"},\"type\":\"ConnectorPlacement.EquallySpacedRectSide\",\"uuid\":\"fdd70777-e9cf-4317-afb6-cae87f75d5b0\"},{\"content\":{\"connectorIds\":[\"RConn1\"],\"side\":\"BOTTOM\"},\"type\":\"ConnectorPlacement.EquallySpacedRectSide\",\"uuid\":\"2353ed68-b1a1-4775-9ca9-31e268d5443b\"}]},\"type\":\"ConnectorPlacement.EquallySpacedConnector\",\"uuid\":\"d5479f4c-4e65-4791-adcb-73df11f88590\"}],\"packageUris\":[\"http://schema.mathworks.com/mf0/Connector/R2020b\"],\"version\":\"1.0\"}"
  mosfet_thermal_4 : Subsystem
      settings: PortSchema="{\"entries\":[{\"content\":{\"sides\":[{\"content\":{\"connectorIds\":[\"LConn1\"]},\"type\":\"ConnectorPlacement.EquallySpacedRectSide\",\"uuid\":\"9277da8d-d460-43e6-8478-dd662f15d226\"},{\"content\":{\"connectorIds\":[],\"side\":\"RIGHT\"},\"type\":\"ConnectorPlacement.EquallySpacedRectSide\",\"uuid\":\"a7ece396-f1d9-4f4f-a05b-db1fc65d6e1d\"},{\"content\":{\"connectorIds\":[\"LConn2\"],\"side\":\"TOP\"},\"type\":\"ConnectorPlacement.EquallySpacedRectSide\",\"uuid\":\"fdd70777-e9cf-4317-afb6-cae87f75d5b0\"},{\"content\":{\"connectorIds\":[\"RConn1\"],\"side\":\"BOTTOM\"},\"type\":\"ConnectorPlacement.EquallySpacedRectSide\",\"uuid\":\"2353ed68-b1a1-4775-9ca9-31e268d5443b\"}]},\"type\":\"ConnectorPlacement.EquallySpacedConnector\",\"uuid\":\"d5479f4c-4e65-4791-adcb-73df11f88590\"}],\"packageUris\":[\"http://schema.mathworks.com/mf0/Connector/R2020b\"],\"version\":\"1.0\"}"
  udc(+) : PMIOPort  Side=Left
  uac(+) : PMIOPort  Port=2  Side=Right
  uac(-) : PMIOPort  Port=3  Side=Right
  udc(-) : PMIOPort  Port=4  Side=Left
  m : Outport
  wires:
  [gate_Q4] -> Bus Creator/28  "gate_cmd_Q4"
  [gate_Q3] -> Bus Creator/27  "gate_cmd_Q3"
  [gate_Q2] -> Bus Creator/26  "gate_cmd_Q2"
  [gate_Q1] -> Bus Creator/25  "gate_cmd_Q1"
  [ic_zvs_Q4] -> Bus Creator/24  "ic_zvs_Q4"
  [ic_zvs_Q3] -> Bus Creator/23  "ic_zvs_Q3"
  [ic_zvs_Q2] -> Bus Creator/22  "ic_zvs_Q2"
  [ic_zvs_Q1] -> Bus Creator/21  "ic_zvs_Q1"
  Bus Creator/1 -> m/1
  [mosfet_HA_temp_Q4] -> Bus Creator/20  "mosfet_HA_temp_Q4"
  [mosfet_JH_temp_Q4] -> Bus Creator/19  "mosfet_JH_temp_Q4"
  [mosfet_current_Q4] -> Bus Creator/18  "mosfet_current_Q4"
  [mosfet_voltage_Q4] -> Bus Creator/17  "mosfet_voltage_Q4"
  [mosfet_ploss_Q4] -> Bus Creator/16  "mosfet_ploss_Q4"
  [mosfet_HA_temp_Q3] -> Bus Creator/15  "mosfet_HA_temp_Q3"
  [mosfet_JH_temp_Q3] -> Bus Creator/14  "mosfet_JH_temp_Q3"
  [mosfet_current_Q3] -> Bus Creator/13  "mosfet_current_Q3"
  [mosfet_voltage_Q3] -> Bus Creator/12  "mosfet_voltage_Q3"
  [mosfet_ploss_Q3] -> Bus Creator/11  "mosfet_ploss_Q3"
  [mosfet_HA_temp_Q2] -> Bus Creator/10  "mosfet_HA_temp_Q2"
  [mosfet_JH_temp_Q2] -> Bus Creator/9  "mosfet_JH_temp_Q2"
  [mosfet_current_Q2] -> Bus Creator/8  "mosfet_current_Q2"
  [mosfet_voltage_Q2] -> Bus Creator/7  "mosfet_voltage_Q2"
  [mosfet_ploss_Q2] -> Bus Creator/6  "mosfet_ploss_Q2"
  [mosfet_HA_temp_Q1] -> Bus Creator/5  "mosfet_HA_temp_Q1"
  [mosfet_JH_temp_Q1] -> Bus Creator/4  "mosfet_JH_temp_Q1"
  [mosfet_current_Q1] -> Bus Creator/3  "mosfet_current_Q1"
  [mosfet_voltage_Q1] -> Bus Creator/2  "mosfet_voltage_Q1"
  [mosfet_ploss_Q1] -> Bus Creator/1  "mosfet_ploss_Q1"
  [gate_Q3] -> Simulink-PS Converter2/1
  Bus Selector/2 -> [gate_Q2]  "<gate_cmd_Q2>"
  Bus Selector/1 -> [gate_Q1]  "<gate_cmd_Q1>"
  Bus Selector/3 -> [gate_Q3]  "<gate_cmd_Q3>"
  [gate_Q4] -> Simulink-PS Converter3/1
  [gate_Q2] -> Simulink-PS Converter1/1
  [gate_Q1] -> Simulink-PS Converter/1
  Bus Selector/4 -> [gate_Q4]  "<gate_cmd_Q4>"
  gate_commands/1 -> Bus Selector/1
  connections:
  mosfet_thermal_1/LConn1 -- Simulink-PS Converter/RConn1
  mosfet_thermal_3/LConn2 -- udc(+)/RConn1 -- mosfet_thermal_1/LConn2
  mosfet_thermal_4/RConn1 -- udc(-)/RConn1 -- mosfet_thermal_2/RConn1
  mosfet_thermal_2/LConn2 -- mosfet_thermal_1/RConn1 -- uac(+)/RConn1
  mosfet_thermal_3/LConn1 -- Simulink-PS Converter2/RConn1
  mosfet_thermal_4/LConn2 -- uac(-)/RConn1 -- mosfet_thermal_3/RConn1
  mosfet_thermal_2/LConn1 -- Simulink-PS Converter1/RConn1
  mosfet_thermal_4/LConn1 -- Simulink-PS Converter3/RConn1

== system sst_cllc_dcx/dcdc_cllc_modA/input_current_control/input_current_control/current_control/iout_ctrl ==
  i_tilde : Inport
  -1 < x < 1 : Saturate  UpperLimit=1  LowerLimit=-1  OutDataTypeStr=double
  1/Ti : Gain  Gain=param.cllc.ctrl.kp_idc  ParamDataTypeStr=double  OutDataTypeStr=double  SaturateOnIntegerOverflow=on
  Sum1 : Sum  Inputs=+++  SaturateOnIntegerOverflow=on
  Sum4 : Sum  Inputs=-+  SaturateOnIntegerOverflow=on
  Unit Delay4 : UnitDelay  SampleTime=-1
  kp2 : Gain  Gain=param.cllc.ctrl.ki_idc*param.glb_time.ts_cllc  ParamDataTypeStr=double  OutDataTypeStr=double  SaturateOnIntegerOverflow=on
  phase_shift : Outport
  wires:
  i_tilde/1 -> kp2/1, 1/Ti/1
  Sum1/1 -> -1 < x < 1/1
  kp2/1 -> Sum1/2
  1/Ti/1 -> Sum1/1, Sum4/1
  Sum4/1 -> Unit Delay4/1
  Unit Delay4/1 -> Sum1/3
  -1 < x < 1/1 -> Sum4/2, phase_shift/1  "phase_shift"

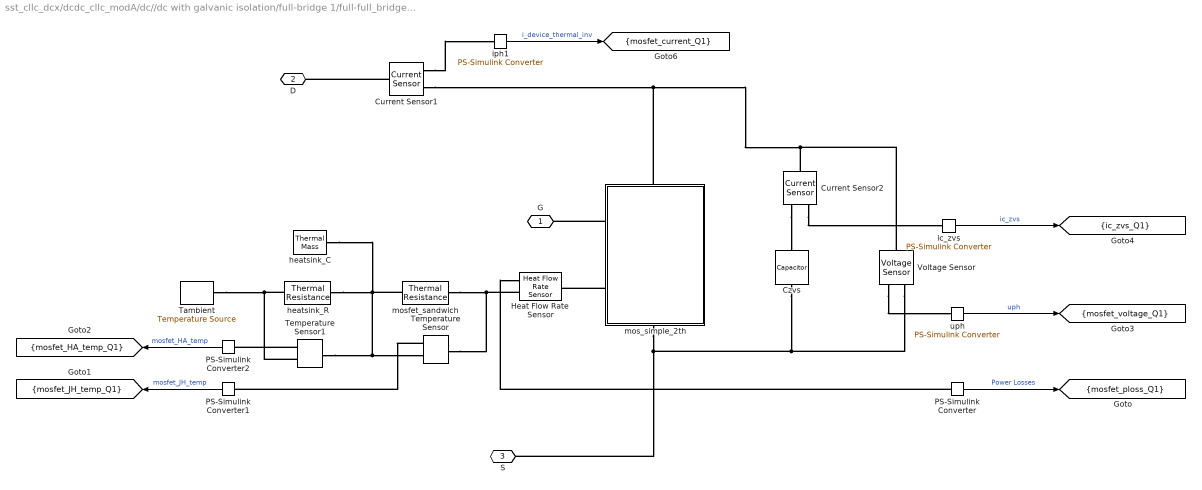
== system sst_cllc_dcx/dcdc_cllc_modA/dc//dc with galvanic isolation/full-bridge 1/full-full_bridge_ssc_mosfet_based/full_bridge_ssc_mosfet_based/mosfet_thermal_1 ==
  Current Sensor1 : fl_lib/Electrical/Electrical Sensors/Current Sensor
  Current Sensor2 : fl_lib/Electrical/Electrical Sensors/Current Sensor
  Czvs : fl_lib/Electrical/Electrical Elements/Capacitor  c=Csnubber_m F  r=Rsnubber_m Ohm  g=0 1/Ohm  i_specify=off  i_priority=None  i=0 A  i_nominal_specify=off  i_nominal_value=1  i_nominal_unit=A  v_specify=off  v_priority=None  v=0 V  v_nominal_specify=off  v_nominal_value=1  v_nominal_unit=V  vc_specify=off  vc_priority=High  vc=0 V  vc_nominal_specify=off  vc_nominal_value=1  vc_nominal_unit=V
  Heat Flow Rate Sensor : fl_lib/Thermal/Thermal Sensors/Heat Flow Rate Sensor
  PS-Simulink Converter : nesl_utility/PS-Simulink Converter  PhysicalDomain=network_engine_domain  SubClassName=ps_output  LeftPortType=input  RightPortType=output  PseudoPeriodic=off  Frequencies=[]  VectorFormat=1-D array  Unit=W  AffineConversion=off
  PS-Simulink Converter1 : nesl_utility/PS-Simulink Converter  PhysicalDomain=network_engine_domain  SubClassName=ps_output  LeftPortType=input  RightPortType=output  PseudoPeriodic=off  Frequencies=[]  VectorFormat=1-D array  Unit=degC  AffineConversion=off
  PS-Simulink Converter2 : nesl_utility/PS-Simulink Converter  PhysicalDomain=network_engine_domain  SubClassName=ps_output  LeftPortType=input  RightPortType=output  PseudoPeriodic=off  Frequencies=[]  VectorFormat=1-D array  Unit=degC  AffineConversion=off
  Tambient : fl_lib/Thermal/Thermal Sources/Temperature Source  temperature=Tambient_m degC
  Temperature Sensor : fl_lib/Thermal/Thermal Sensors/Temperature Sensor  temperature_measure=foundation.enum.MeasurementReference.difference
  Temperature Sensor1 : fl_lib/Thermal/Thermal Sensors/Temperature Sensor  temperature_measure=foundation.enum.MeasurementReference.difference
  Voltage Sensor : fl_lib/Electrical/Electrical Sensors/Voltage Sensor
  heatsink_C : fl_lib/Thermal/Thermal Elements/Thermal Mass  mass_type=foundation.enum.constant_variable.constant  mass=mass_heatsink_m kg  sp_heat=specific_heat_m J/(K*kg)  mass_min=1e-6 kg  num_ports=foundation.enum.numPorts2.one  m_specify=off  m_priority=High  m=1 kg  m_nominal_specify=off  m_nominal_value=1  m_nominal_unit=kg  T_specify=on  T_priority=High  T=DThs_init_m+Tambient_m degC  T_nominal_specify=off  T_nominal_value=1  T_nominal_unit=K  Q_specify=off  Q_priority=High  Q=0 W  Q_nominal_specify=off  Q_nominal_value=1  Q_nominal_unit=W
  heatsink_R : fl_lib/Thermal/Thermal Elements/Thermal Resistance  resistance=rth_mosfet_HA_m K/W  T_specify=off  T_priority=High  T=0 deltadegC  T_nominal_specify=off  T_nominal_value=1  T_nominal_unit=K  Q_specify=off  Q_priority=None  Q=0 W  Q_nominal_specify=off  Q_nominal_value=1  Q_nominal_unit=W
  ic_zvs : nesl_utility/PS-Simulink Converter  PhysicalDomain=network_engine_domain  SubClassName=ps_output  LeftPortType=input  RightPortType=output  PseudoPeriodic=off  Frequencies=[]  VectorFormat=1-D array  Unit=A  AffineConversion=off
  iph1 : nesl_utility/PS-Simulink Converter  PhysicalDomain=network_engine_domain  SubClassName=ps_output  LeftPortType=input  RightPortType=output  PseudoPeriodic=off  Frequencies=[]  VectorFormat=1-D array  Unit=A  AffineConversion=off
  mos_simple_2th : Subsystem
      settings: PortSchema="{\"entries\":[{\"content\":{\"sides\":[{\"content\":{\"connectorIds\":[\"LConn1\",\"LConn2\"]},\"type\":\"ConnectorPlacement.EquallySpacedRectSide\",\"uuid\":\"0c7df1d1-e739-4cca-908e-e4e85a8d5110\"},{\"content\":{\"side\":\"RIGHT\"},\"type\":\"ConnectorPlacement.EquallySpacedRectSide\",\"uuid\":\"6e0178b8-4891-4b94-aab6-d38b52a6c94b\"},{\"content\":{\"connectorIds\":[\"LConn3\"],\"side\":\"TOP\"},\"type\":\"ConnectorPlacement.EquallySpacedRectSide\",\"uuid\":\"66a82ce3-a212-45ef-89fa-79c9554ad3a2\"},{\"content\":{\"connectorIds\":[\"RConn1\"],\"side\":\"BOTTOM\"},\"type\":\"ConnectorPlacement.EquallySpacedRectSide\",\"uuid\":\"30e3dab1-9356-4de4-b881-b8bc9cf47aa5\"}]},\"type\":\"ConnectorPlacement.EquallySpacedConnector\",\"uuid\":\"69805b64-ad78-46b1-90c4-7e7bc5808829\"}],\"packageUris\":[\"http://schema.mathworks.com/mf0/Connector/R2020b\"],\"version\":\"1.0\"}"
  mosfet_sandwich : fl_lib/Thermal/Thermal Elements/Thermal Resistance  resistance=rth_mosfet_JH_m K/W  T_specify=off  T_priority=High  T=0 degC  T_nominal_specify=off  T_nominal_value=1  T_nominal_unit=K  Q_specify=off  Q_priority=None  Q=0 W  Q_nominal_specify=off  Q_nominal_value=1  Q_nominal_unit=W
  uph : nesl_utility/PS-Simulink Converter  PhysicalDomain=network_engine_domain  SubClassName=ps_output  LeftPortType=input  RightPortType=output  PseudoPeriodic=off  Frequencies=[]  VectorFormat=1-D array  Unit=V  AffineConversion=off
  G : PMIOPort  Side=Left
  D : PMIOPort  Port=2  Side=Left
  S : PMIOPort  Port=3  Side=Right
  tag scope: ic_zvs_Q1=scoped, mosfet_HA_temp_Q1=scoped, mosfet_JH_temp_Q1=scoped, mosfet_current_Q1=scoped, mosfet_ploss_Q1=scoped, mosfet_voltage_Q1=scoped
  wires:
  ic_zvs/1 -> [ic_zvs_Q1]  "ic_zvs"
  uph/1 -> [mosfet_voltage_Q1]  "uph"
  iph1/1 -> [mosfet_current_Q1]  "i_device_thermal_inv"
  PS-Simulink Converter1/1 -> [mosfet_JH_temp_Q1]  "mosfet_JH_temp"
  PS-Simulink Converter2/1 -> [mosfet_HA_temp_Q1]  "mosfet_HA_temp"
  PS-Simulink Converter/1 -> [mosfet_ploss_Q1]  "Power Losses"
  connections:
  Current Sensor2/RConn1 -- ic_zvs/LConn1
  Current Sensor2/RConn2 -- Czvs/LConn1
  Voltage Sensor/RConn1 -- uph/LConn1
  Current Sensor1/RConn1 -- iph1/LConn1
  Voltage Sensor/LConn1 -- mos_simple_2th/LConn3 -- Current Sensor1/RConn2 -- Current Sensor2/LConn1
  Current Sensor1/LConn1 -- D/RConn1
  mos_simple_2th/LConn2 -- Heat Flow Rate Sensor/LConn1
  Temperature Sensor1/RConn2 -- PS-Simulink Converter2/LConn1
  Temperature Sensor1/RConn1 -- heatsink_R/RConn1 -- Tambient/LConn1
  Temperature Sensor/RConn2 -- PS-Simulink Converter1/LConn1
  heatsink_C/LConn1 -- heatsink_R/LConn1 -- mosfet_sandwich/RConn1 -- Temperature Sensor/RConn1 -- Temperature Sensor1/LConn1
  Heat Flow Rate Sensor/RConn2 -- mosfet_sandwich/LConn1 -- Temperature Sensor/LConn1
  PS-Simulink Converter/LConn1 -- Heat Flow Rate Sensor/RConn1
  mos_simple_2th/LConn1 -- G/RConn1
  Voltage Sensor/RConn2 -- Czvs/RConn1 -- mos_simple_2th/RConn1 -- S/RConn1

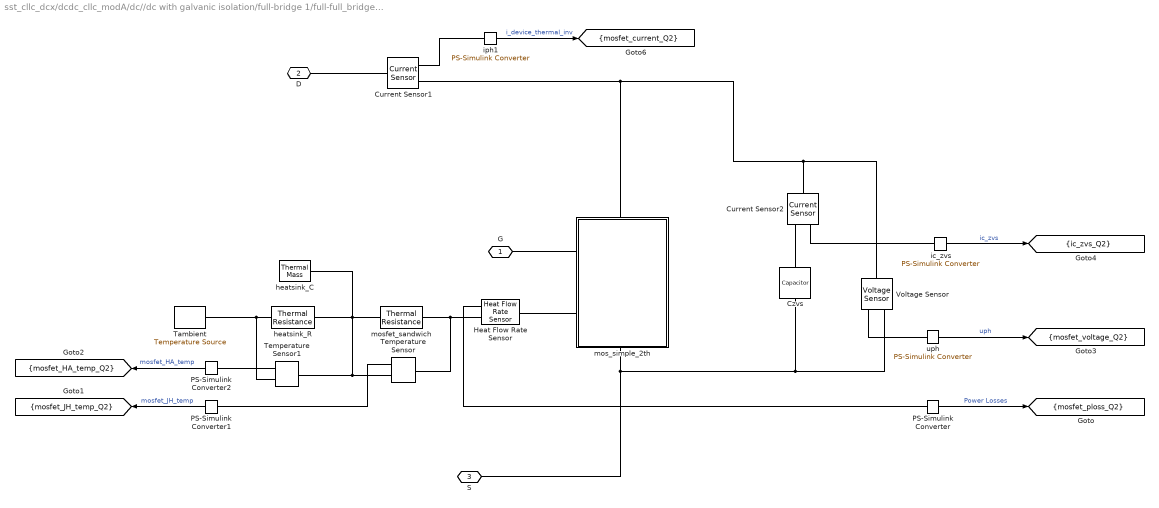
== system sst_cllc_dcx/dcdc_cllc_modA/dc//dc with galvanic isolation/full-bridge 1/full-full_bridge_ssc_mosfet_based/full_bridge_ssc_mosfet_based/mosfet_thermal_2 ==
  Current Sensor1 : fl_lib/Electrical/Electrical Sensors/Current Sensor
  Current Sensor2 : fl_lib/Electrical/Electrical Sensors/Current Sensor
  Czvs : fl_lib/Electrical/Electrical Elements/Capacitor  c=Csnubber_m F  r=Rsnubber_m Ohm  g=0 1/Ohm  i_specify=off  i_priority=None  i=0 A  i_nominal_specify=off  i_nominal_value=1  i_nominal_unit=A  v_specify=off  v_priority=None  v=0 V  v_nominal_specify=off  v_nominal_value=1  v_nominal_unit=V  vc_specify=off  vc_priority=High  vc=0 V  vc_nominal_specify=off  vc_nominal_value=1  vc_nominal_unit=V
  Heat Flow Rate Sensor : fl_lib/Thermal/Thermal Sensors/Heat Flow Rate Sensor
  PS-Simulink Converter : nesl_utility/PS-Simulink Converter  PhysicalDomain=network_engine_domain  SubClassName=ps_output  LeftPortType=input  RightPortType=output  PseudoPeriodic=off  Frequencies=[]  VectorFormat=1-D array  Unit=W  AffineConversion=off
  PS-Simulink Converter1 : nesl_utility/PS-Simulink Converter  PhysicalDomain=network_engine_domain  SubClassName=ps_output  LeftPortType=input  RightPortType=output  PseudoPeriodic=off  Frequencies=[]  VectorFormat=1-D array  Unit=degC  AffineConversion=off
  PS-Simulink Converter2 : nesl_utility/PS-Simulink Converter  PhysicalDomain=network_engine_domain  SubClassName=ps_output  LeftPortType=input  RightPortType=output  PseudoPeriodic=off  Frequencies=[]  VectorFormat=1-D array  Unit=degC  AffineConversion=off
  Tambient : fl_lib/Thermal/Thermal Sources/Temperature Source  temperature=Tambient_m degC
  Temperature Sensor : fl_lib/Thermal/Thermal Sensors/Temperature Sensor  temperature_measure=foundation.enum.MeasurementReference.difference
  Temperature Sensor1 : fl_lib/Thermal/Thermal Sensors/Temperature Sensor  temperature_measure=foundation.enum.MeasurementReference.difference
  Voltage Sensor : fl_lib/Electrical/Electrical Sensors/Voltage Sensor
  heatsink_C : fl_lib/Thermal/Thermal Elements/Thermal Mass  mass_type=foundation.enum.constant_variable.constant  mass=mass_heatsink_m kg  sp_heat=specific_heat_m J/(K*kg)  mass_min=1e-6 kg  num_ports=foundation.enum.numPorts2.one  m_specify=off  m_priority=High  m=1 kg  m_nominal_specify=off  m_nominal_value=1  m_nominal_unit=kg  T_specify=on  T_priority=High  T=DThs_init_m+Tambient_m degC  T_nominal_specify=off  T_nominal_value=1  T_nominal_unit=K  Q_specify=off  Q_priority=High  Q=0 W  Q_nominal_specify=off  Q_nominal_value=1  Q_nominal_unit=W
  heatsink_R : fl_lib/Thermal/Thermal Elements/Thermal Resistance  resistance=rth_mosfet_HA_m K/W  T_specify=off  T_priority=High  T=0 deltadegC  T_nominal_specify=off  T_nominal_value=1  T_nominal_unit=K  Q_specify=off  Q_priority=None  Q=0 W  Q_nominal_specify=off  Q_nominal_value=1  Q_nominal_unit=W
  ic_zvs : nesl_utility/PS-Simulink Converter  PhysicalDomain=network_engine_domain  SubClassName=ps_output  LeftPortType=input  RightPortType=output  PseudoPeriodic=off  Frequencies=[]  VectorFormat=1-D array  Unit=A  AffineConversion=off
  iph1 : nesl_utility/PS-Simulink Converter  PhysicalDomain=network_engine_domain  SubClassName=ps_output  LeftPortType=input  RightPortType=output  PseudoPeriodic=off  Frequencies=[]  VectorFormat=1-D array  Unit=A  AffineConversion=off
  mos_simple_2th : Subsystem
      settings: PortSchema="{\"entries\":[{\"content\":{\"sides\":[{\"content\":{\"connectorIds\":[\"LConn1\",\"LConn2\"]},\"type\":\"ConnectorPlacement.EquallySpacedRectSide\",\"uuid\":\"0c7df1d1-e739-4cca-908e-e4e85a8d5110\"},{\"content\":{\"side\":\"RIGHT\"},\"type\":\"ConnectorPlacement.EquallySpacedRectSide\",\"uuid\":\"6e0178b8-4891-4b94-aab6-d38b52a6c94b\"},{\"content\":{\"connectorIds\":[\"LConn3\"],\"side\":\"TOP\"},\"type\":\"ConnectorPlacement.EquallySpacedRectSide\",\"uuid\":\"66a82ce3-a212-45ef-89fa-79c9554ad3a2\"},{\"content\":{\"connectorIds\":[\"RConn1\"],\"side\":\"BOTTOM\"},\"type\":\"ConnectorPlacement.EquallySpacedRectSide\",\"uuid\":\"30e3dab1-9356-4de4-b881-b8bc9cf47aa5\"}]},\"type\":\"ConnectorPlacement.EquallySpacedConnector\",\"uuid\":\"69805b64-ad78-46b1-90c4-7e7bc5808829\"}],\"packageUris\":[\"http://schema.mathworks.com/mf0/Connector/R2020b\"],\"version\":\"1.0\"}"
  mosfet_sandwich : fl_lib/Thermal/Thermal Elements/Thermal Resistance  resistance=rth_mosfet_JH_m K/W  T_specify=off  T_priority=High  T=0 degC  T_nominal_specify=off  T_nominal_value=1  T_nominal_unit=K  Q_specify=off  Q_priority=None  Q=0 W  Q_nominal_specify=off  Q_nominal_value=1  Q_nominal_unit=W
  uph : nesl_utility/PS-Simulink Converter  PhysicalDomain=network_engine_domain  SubClassName=ps_output  LeftPortType=input  RightPortType=output  PseudoPeriodic=off  Frequencies=[]  VectorFormat=1-D array  Unit=V  AffineConversion=off
  G : PMIOPort  Side=Left
  D : PMIOPort  Port=2  Side=Left
  S : PMIOPort  Port=3  Side=Right
  tag scope: ic_zvs_Q2=scoped, mosfet_HA_temp_Q2=scoped, mosfet_JH_temp_Q2=scoped, mosfet_current_Q2=scoped, mosfet_ploss_Q2=scoped, mosfet_voltage_Q2=scoped
  wires:
  ic_zvs/1 -> [ic_zvs_Q2]  "ic_zvs"
  PS-Simulink Converter/1 -> [mosfet_ploss_Q2]  "Power Losses"
  PS-Simulink Converter2/1 -> [mosfet_HA_temp_Q2]  "mosfet_HA_temp"
  PS-Simulink Converter1/1 -> [mosfet_JH_temp_Q2]  "mosfet_JH_temp"
  iph1/1 -> [mosfet_current_Q2]  "i_device_thermal_inv"
  uph/1 -> [mosfet_voltage_Q2]  "uph"
  connections:
  Current Sensor2/RConn1 -- ic_zvs/LConn1
  Czvs/LConn1 -- Current Sensor2/RConn2
  Czvs/RConn1 -- mos_simple_2th/RConn1 -- S/RConn1 -- Voltage Sensor/RConn2
  mos_simple_2th/LConn1 -- G/RConn1
  PS-Simulink Converter/LConn1 -- Heat Flow Rate Sensor/RConn1
  Temperature Sensor/LConn1 -- mosfet_sandwich/LConn1 -- Heat Flow Rate Sensor/RConn2
  heatsink_R/LConn1 -- heatsink_C/LConn1 -- mosfet_sandwich/RConn1 -- Temperature Sensor/RConn1 -- Temperature Sensor1/LConn1
  Temperature Sensor/RConn2 -- PS-Simulink Converter1/LConn1
  Tambient/LConn1 -- heatsink_R/RConn1 -- Temperature Sensor1/RConn1
  Temperature Sensor1/RConn2 -- PS-Simulink Converter2/LConn1
  mos_simple_2th/LConn2 -- Heat Flow Rate Sensor/LConn1
  Current Sensor1/LConn1 -- D/RConn1
  Current Sensor2/LConn1 -- Voltage Sensor/LConn1 -- mos_simple_2th/LConn3 -- Current Sensor1/RConn2
  Current Sensor1/RConn1 -- iph1/LConn1
  Voltage Sensor/RConn1 -- uph/LConn1
